simulink subsystem "Aero_RW"  (R2025a)
settings: Solver=VariableStepAuto  StartTime=0.0  StopTime=10.0  RelTol=1e-3
undefined symbols (not defined in the file or in its folder): HIL
libraries: quarc_library x3
settings Model: Creator=najem1u  LastModifiedBy=rayan

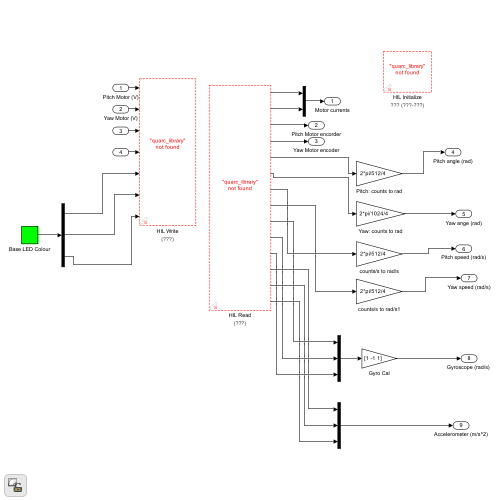
[thumbnail: Simulink's stored preview of the top-level diagram]
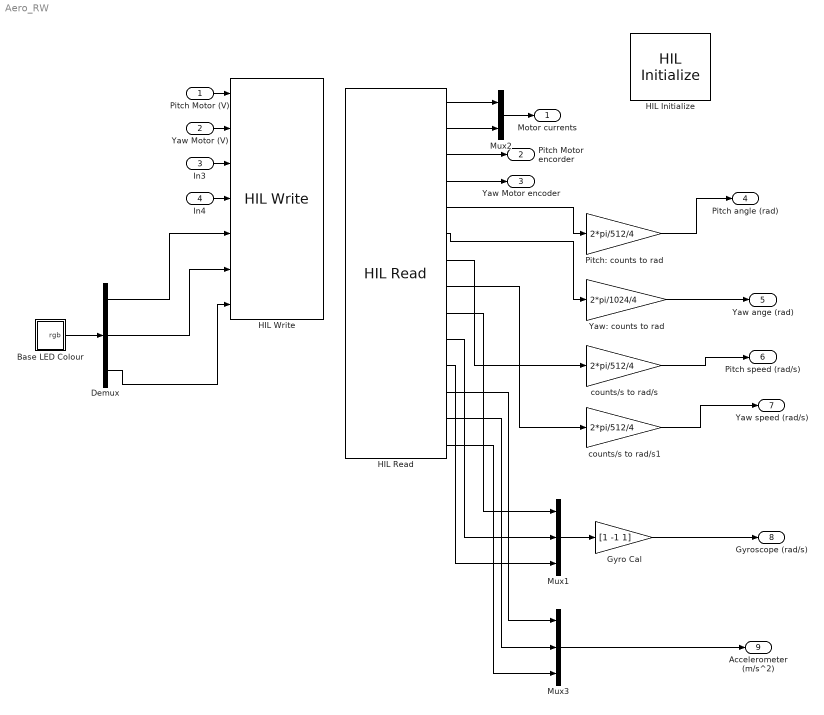
== system Aero_RW ==
  Pitch Motor (V) : Inport
  Yaw Motor (V) : Inport  Port=2
  In3 : Inport  Port=3
  In4 : Inport  Port=4
  Base LED Colour : Subsystem  mask(Color Constant){color=[0 1 0]}
      mask help: Outputs a constant RGB color value.
      mask init:
      | rgb = get_param(gcbh, 'color');
      | if numel(color) ~= 3
      |     rgb = [0 0 0];
      | end
      | set_param(gcbh, 'MaskDisplay', ['patch([-0.02 -0.02 1.02 1.02], [-0.02 1.02 1.02 -0.02], ', rgb, ');']);
      settings: OpenFcn=color_constant_properties('CurrentBlock', gcbh);
      mask Help: web(qc_get_block_help_path(gcb), '-helpbrowser');
      mask Display: patch([-0.02 -0.02 1.02 1.02], [-0.02 1.02 1.02 -0.02], [0 1 0]);
  Demux : Demux  Outputs=3
  Gyro Cal : Gain  Gain=[1 -1 1]
  HIL Initialize : quarc_library/Data Acquisition/Generic/Configuration/HIL Initialize  object_name=HIL-1  board_type=quanser_aero_usb  board_number=0  board_options=""  exclusive=off  active=on  hardware_clocks=[0]  clock_modes=[]  initial_clock_frequencies=[]  set_clock_params_at_start=off  set_clock_params_at_switch_in=off  set_clock_frequencies_at_start=off  set_clock_frequencies_at_switch_in=off  analog_input_channels=[0:1]  analog_input_configurations=[]  analog_input_maximums=3  analog_input_minimums=-3  set_analog_input_params_at_start=off  set_analog_input_params_at_switch_in=off  analog_output_channels=[0:1]  analog_output_maximums=24  analog_output_minimums=-24  initial_analog_outputs=[0]  final_analog_outputs=[0]  watchdog_analog_outputs=[0]  set_analog_output_params_at_start=off  set_analog_output_params_at_switch_in=off  set_analog_outputs_at_start=on  set_analog_outputs_at_switch_in=off  set_analog_outputs_at_terminate=on  set_analog_outputs_at_switch_out=off  set_analog_outputs_on_watchdog=on  digital_input_channels=[]  digital_output_channels=[0:1]  digital_output_configuration=[]  initial_digital_outputs=[1]  final_digital_outputs=[0]  watchdog_digital_outputs=[0]  set_digital_output_params_at_start=off  set_digital_output_params_at_switch_in=off  set_digital_outputs_at_start=on  set_digital_outputs_at_switch_in=off  set_digital_outputs_at_terminate=on  set_digital_outputs_at_switch_out=off  set_digital_outputs_on_watchdog=on  encoder_channels=[0:3]  quadrature=[4]  encoder_filter_frequency=[]  initial_encoder_counts=[0]  set_encoder_params_at_start=off  set_encoder_params_at_switch_in=off  set_encoder_counts_at_start=on  set_encoder_counts_at_switch_in=off  pwm_channels=[]  pwm_modes=[]  pwm_frequency=[]  pwm_configuration=[]  pwm_alignment=[]  pwm_polarity=[]  pwm_leading_deadband=[]  pwm_trailing_deadband=[]  initial_pwm_outputs=[]  final_pwm_outputs=[]  watchdog_pwm_outputs=[]  set_pwm_params_at_start=off  set_pwm_params_at_switch_in=off  set_pwm_outputs_at_start=off  set_pwm_outputs_at_switch_in=off  set_pwm_outputs_at_terminate=off  set_pwm_outputs_at_switch_out=off  set_pwm_outputs_on_watchdog=off  other_output_channels=[11000:11002]  initial_other_outputs=[0 1 0]  final_other_outputs=[1 0 0]  watchdog_other_outputs=[0 0 1]  set_other_outputs_at_start=on  set_other_outputs_at_switch_in=off  set_other_outputs_at_terminate=on  set_other_outputs_at_switch_out=off  set_other_outputs_on_watchdog=on
  HIL Read : quarc_library/Data Acquisition/Generic/Immediate I//O/HIL Read  object_name=HIL-1  analog_channels=[0:1]  encoder_channels=[0:3]  digital_channels=[]  other_channels=[14000:14001 3000:3002 4000:4002]  sample_time=qc_get_step_size  active=on  vector_output=off  data_type_mode=Inherit via back propagation  encoder_data_type=double  digital_data_type=boolean
  HIL Write : quarc_library/Data Acquisition/Generic/Immediate I//O/HIL Write  object_name=HIL-1  analog_channels=[0:1]  pwm_channels=[]  digital_channels=[0:1]  other_channels=[11000:11002]  sample_time=-1  active=off  vector_input=off
  Mux1 : Mux  Inputs=3
  Mux2 : Mux  Inputs=2
  Mux3 : Mux  Inputs=3
  Pitch: counts to rad : Gain  Gain=2*pi/512/4
  Yaw: counts to rad : Gain  Gain=2*pi/1024/4
  counts/s to rad/s : Gain  Gain=2*pi/512/4
  counts/s to rad/s1 : Gain  Gain=2*pi/512/4
  Motor currents : Outport
  Pitch Motor encorder : Outport  Port=2
  Yaw Motor encoder : Outport  Port=3
  Pitch angle (rad) : Outport  Port=4
  Yaw ange (rad) : Outport  Port=5
  Pitch speed (rad/s) : Outport  Port=6
  Yaw speed (rad/s) : Outport  Port=7
  "Gyroscope (rad/s) " : Outport  Port=8
  Accelerometer (m/s^2) : Outport  Port=9
  wires:
  HIL Read/3 -> Pitch Motor encorder/1
  HIL Read/2 -> Mux2/2
  Demux/2 -> HIL Write/6
  Pitch Motor (V)/1 -> HIL Write/1
  HIL Read/4 -> Yaw Motor encoder/1
  Yaw Motor (V)/1 -> HIL Write/2
  In3/1 -> HIL Write/3
  In4/1 -> HIL Write/4
  Demux/1 -> HIL Write/5
  Demux/3 -> HIL Write/7
  Base LED Colour/1(rgb) -> Demux/1
  HIL Read/5 -> Pitch: counts to rad/1
  HIL Read/6 -> Yaw: counts to rad/1
  HIL Read/7 -> counts/s to rad/s/1
  HIL Read/8 -> counts/s to rad/s1/1
  Pitch: counts to rad/1 -> Pitch angle (rad)/1
  counts/s to rad/s1/1 -> Yaw speed (rad/s)/1
  counts/s to rad/s/1 -> Pitch speed (rad/s)/1
  Yaw: counts to rad/1 -> Yaw ange (rad)/1
  Mux1/1 -> Gyro Cal/1
  HIL Read/9 -> Mux1/1
  HIL Read/10 -> Mux1/2
  HIL Read/11 -> Mux1/3
  HIL Read/12 -> Mux3/1
  HIL Read/13 -> Mux3/2
  HIL Read/14 -> Mux3/3
  Gyro Cal/1 -> "Gyroscope (rad/s) "/1
  Mux3/1 -> Accelerometer (m/s^2)/1
  HIL Read/1 -> Mux2/1
  Mux2/1 -> Motor currents/1

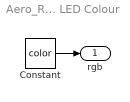
== system Aero_RW/Base LED Colour ==
  Constant : Constant  Value=color
  rgb : Outport
  wires:
  Constant/1 -> rgb/1
